simulink subsystem "rb2_sensor_reference"  (R2024b)
settings: Solver=VariableStepAuto  StartTime=0.0  StopTime=10.0  RelTol=1e-3
values from neighbouring files (symbols this model uses):
  cfg = testbench_config()    [export_robot_geometry.m]
undefined symbols (not defined in the file or in its folder): aButter, alpha, bButter, bias_est
libraries: simulink x1
settings Model: Creator=pc  LastModifiedBy=pc

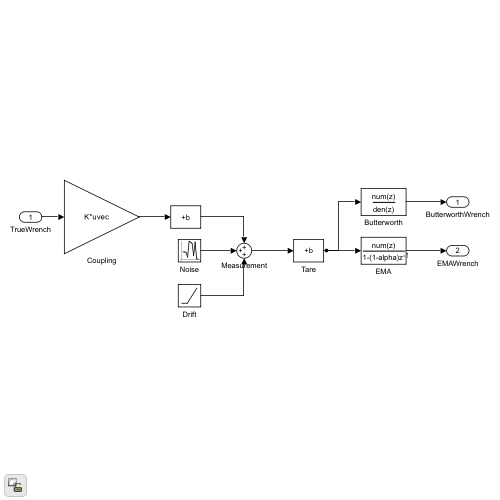
[thumbnail: Simulink's stored preview of the top-level diagram]
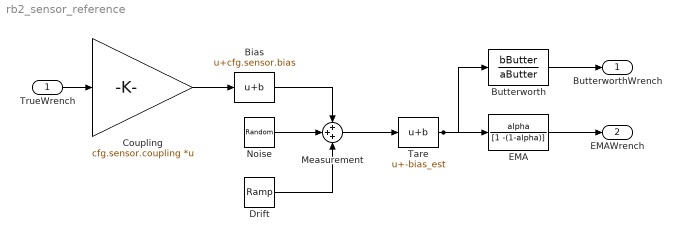
== system rb2_sensor_reference ==
  TrueWrench : Inport
  Bias : Bias  Bias=cfg.sensor.bias  SaturateOnIntegerOverflow=off
  Butterworth : DiscreteFilter  Numerator=bButter  Denominator=aButter
  Coupling : Gain  Gain=cfg.sensor.coupling  Multiplication=Matrix(K*u) (u vector)
  Drift : simulink/Sources/Ramp  slope=cfg.sensor.drift_per_s  start=0  InitialOutput=zeros(6,1)
  EMA : DiscreteFilter  Numerator=alpha  Denominator=[1 -(1-alpha)]
  Measurement : Sum  Inputs=+++
  Noise : RandomNumber  Mean=zeros(6,1)  Variance=cfg.sensor.noise_std.^2  Seed=[17;18;19;20;21;22]  SampleTime=.002
  Tare : Bias  Bias=-bias_est  SaturateOnIntegerOverflow=off
  ButterworthWrench : Outport
  EMAWrench : Outport  Port=2
  wires:
  Butterworth/1 -> ButterworthWrench/1
  EMA/1 -> EMAWrench/1
  TrueWrench/1 -> Coupling/1
  Bias/1 -> Measurement/1
  Noise/1 -> Measurement/2
  Coupling/1 -> Bias/1
  Drift/1 -> Measurement/3
  Measurement/1 -> Tare/1
  Tare/1 -> Butterworth/1, EMA/1
